simulink model "CAP"  (Simulink 10.0)
settings: Solver=ode45  StartTime=0.0  StopTime=inf  RelTol=1e-3  EnableMultiTasking=on
InitFcn:
  | wt = 0:2*pi/30:4*pi;   % time axis for pulse generation
  | 
  | g = rcosine(1,10);      % raised cosine as chosen pulse
  | 
  | inphase_pulse = g .* cos(wt);      % in-phase pulse
  | quadrature_pulse = g .* sin(wt);   % quadrature pulse
libraries: commdigbbndam2 x2, commchan2 x1, commrandsrc2 x1
settings Model: Creator=chiha  LastModifiedBy=chiha
settings DataIOCC: LimitDataPoints=on  SignalLoggingSaveFormat=ModelDataLogs
settings OptimizationCC: InitFltsAndDblsToZero=on
settings DebuggingCC: SaveWithParameterizedLinksMsg=none  SignalResolutionControl=TryResolveAllWithWarning  SolverPrmCheckMsg=warning  MultiTaskDSMMsg=warning  MultiTaskCondExecSysMsg=none
settings ModelReferenceCC: EnableRefExpFcnMdlSchedulingChecks=off
settings SFSimCC: SimUseLocalCustomCode=on  CustomCodeUndefinedFunction=FilterOut
settings RTWCC: RTWUseLocalCustomCode=on
settings GRTTargetCC: TargetFcnLib=ansi_tfl_tmw.mat

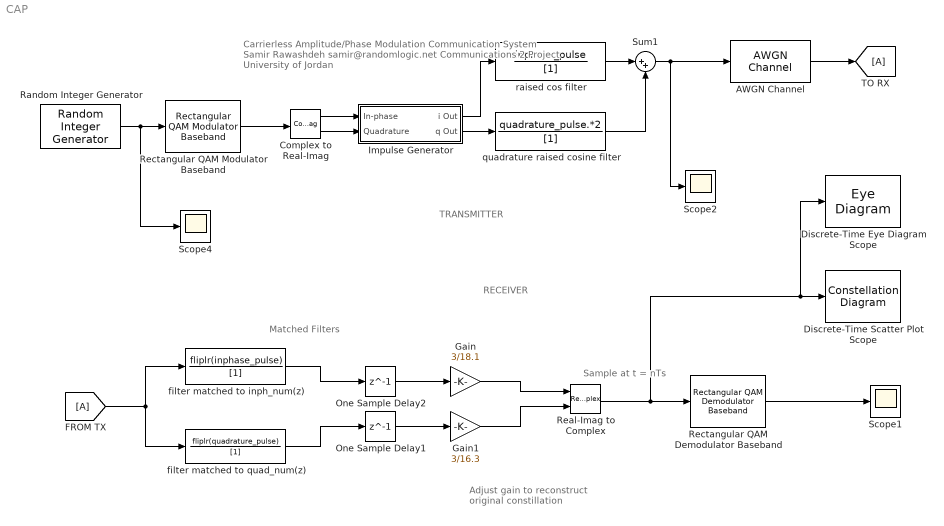
== system CAP ==
  note: Carrierless Amplitude/Phase Modulation Communication System
      | Samir Rawashdeh
      | samir@randomlogic.net
      | Communications 2 Project
      | University of Jordan
  note: TRANSMITTER
  note: RECEIVER
  note: Matched Filters
  note: Adjust gain to reconstruct
      | original constillation
  note: Sample at t = nTs
  AWGN Channel : commchan2/AWGN Channel  seed=67  noiseMode="Signal to noise ratio  (Eb/No)"  EbNodB=7  EsNodB=10  SNRdB=10  bitsPerSym=1  Ps=1  Tsym=1  variance=1
  Complex to Real-Imag : ComplexToRealImag
  Discrete-Time Eye Diagram Scope : EyeDiagram  Tag=EyeDiagram  DefaultConfigurationName=comm.scopes.EyeDiagramBlockCfg
  Discrete-Time Scatter Plot Scope : ConstellationDiagram  Tag=ScatterPlot  DefaultConfigurationName=comm.scopes.ConstellationDiagramBlockCfg  FigPos=[296 204 560 560]
  Gain : Gain  Gain=3/18.1
  Gain1 : Gain  Gain=3/16.3
  Impulse Generator : Subsystem
  One Sample Delay1 : Delay  DelayLength=1
  One Sample Delay2 : Delay  DelayLength=1
  Random Integer Generator : commrandsrc2/Random Integer Generator  mul=16  seed=37  Ts=length(wt)  frameBased=off  sampPerFrame=1  orient=off
  Real-Imag to Complex : RealImagToComplex  SampleTime=length(wt)
  Rectangular QAM Demodulator Baseband : commdigbbndam2/Rectangular QAM Demodulator Baseband  M=16  OutType=Integer  Dec=Binary  PowType=Min. distance between symbols  MinDist=2  AvgPow=1  PeakPow=1  Ph=0  numSamp=1
  Rectangular QAM Modulator Baseband : commdigbbndam2/Rectangular QAM Modulator Baseband  M=16  InType=Integer  Enc=Binary  PowType=Min. distance between symbols  MinDist=2  AvgPow=1  PeakPow=1  Ph=0  numSamp=1
  Scope1 : Scope
  Scope2 : Scope
  Scope4 : Scope
  Sum1 : Sum  Inputs=|++
  filter matched to inph_num(z) : DiscreteFilter  Numerator=fliplr(inphase_pulse)  Denominator=[1]  SampleTime=1
  filter matched to quad_num(z) : DiscreteFilter  Numerator=fliplr(quadrature_pulse)  Denominator=[1]  SampleTime=1
  quadrature raised cosine filter : DiscreteFilter  Numerator=quadrature_pulse.*2  Denominator=[1]  SampleTime=1
  raised cos filter : DiscreteFilter  Numerator=inphase_pulse  Denominator=[1]  SampleTime=1
  wires:
  Rectangular QAM Modulator Baseband/1 -> Complex to Real-Imag/1
  quadrature raised cosine filter/1 -> Sum1/2
  raised cos filter/1 -> Sum1/1
  Complex to Real-Imag/1 -> Impulse Generator/1(In-phase)
  Complex to Real-Imag/2 -> Impulse Generator/2(Quadrature)
  Impulse Generator/1(i Out) -> raised cos filter/1
  Impulse Generator/2(q Out) -> quadrature raised cosine filter/1
  [A] -> filter matched to quad_num(z)/1, filter matched to inph_num(z)/1
  filter matched to inph_num(z)/1 -> One Sample Delay2/1
  filter matched to quad_num(z)/1 -> One Sample Delay1/1
  One Sample Delay2/1 -> Gain/1
  One Sample Delay1/1 -> Gain1/1
  Sum1/1 -> AWGN Channel/1, Scope2/1
  AWGN Channel/1 -> [A]
  Random Integer Generator/1 -> Rectangular QAM Modulator Baseband/1, Scope4/1
  Gain/1 -> Real-Imag to Complex/1
  Gain1/1 -> Real-Imag to Complex/2
  Rectangular QAM Demodulator Baseband/1 -> Scope1/1
  Real-Imag to Complex/1 -> Rectangular QAM Demodulator Baseband/1, Discrete-Time Scatter Plot Scope/1, Discrete-Time Eye Diagram Scope/1

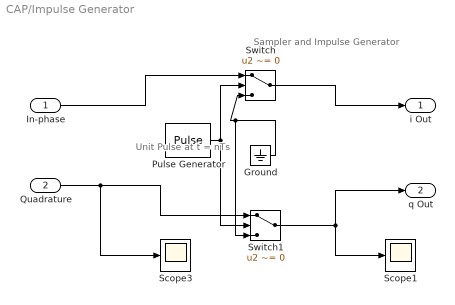
== system CAP/Impulse Generator ==
  note: Unit Pulse
      | at t = nTs
  note: Sampler and Impulse Generator
  In-phase : Inport
  Quadrature : Inport  Port=2
  Ground : Ground
  Pulse Generator : DiscretePulseGenerator  Period=length(wt)
  Scope1 : Scope
  Scope3 : Scope
  Switch : Switch  Criteria=u2 ~= 0
  Switch1 : Switch  Criteria=u2 ~= 0
  i Out : Outport
  q Out : Outport  Port=2
  wires:
  Pulse Generator/1 -> Switch/2, Switch1/2
  Ground/1 -> Switch/3, Switch1/3
  In-phase/1 -> Switch/1
  Quadrature/1 -> Switch1/1, Scope3/1
  Switch/1 -> i Out/1
  Switch1/1 -> q Out/1, Scope1/1
